simulink model "fs_driverless_top"  (R2026b)
settings: Solver=FixedStepDiscrete  StopTime=P.tEnd  FixedStep=P.dt
undefined symbols (not defined in the file): cones, lidarCfg, P, perception
libraries: sim3dlib x2, sim3dphyssensorlib x1, sim3dautolib x1
settings Model: Creator=User  LastModifiedBy=Jun Yee

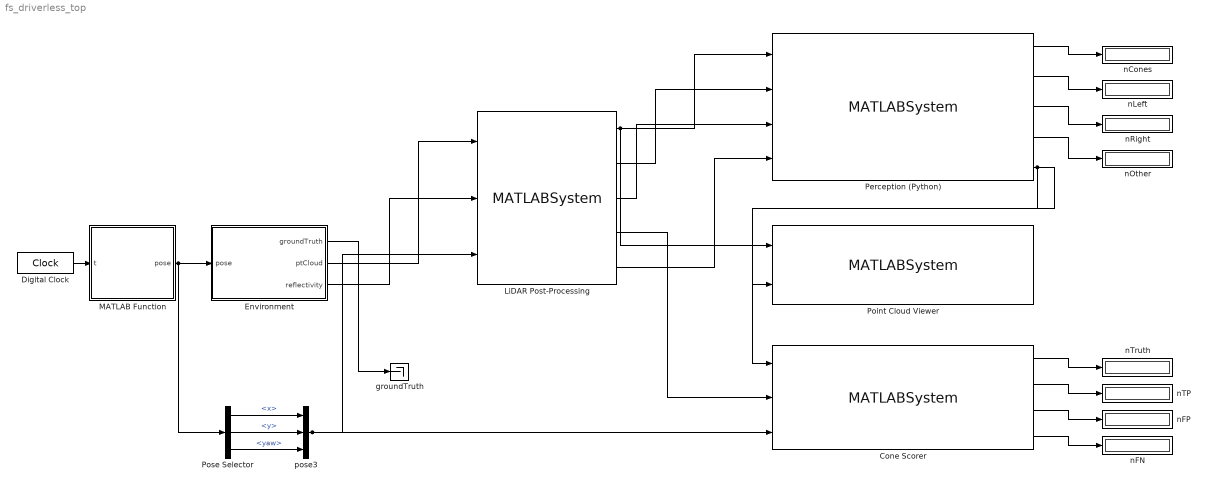
== system fs_driverless_top ==
  Cone Scorer : MATLABSystem  System=ConeScorer  MaxRange=P.score.maxRange  Gate=P.score.gate  MinHits=P.score.minHits  SensorOffset=lidarCfg.refToSensor  Ts=lidarCfg.Ts  PoseLag=lidarCfg.poseLagScans  SimulateUsing=Interpreted execution
      mask Type: ConeScorer
  Digital Clock : DigitalClock  SampleTime=P.dt
  Environment : Subsystem
  LiDAR Post-Processing : MATLABSystem  System=LidarPostProcess  MinRange=lidarCfg.minRange  MaxRange=lidarCfg.range  NoiseStd=lidarCfg.noiseStd  Ts=lidarCfg.Ts  Az=lidarCfg.az  ScanStartAz=lidarCfg.scanStartAz  SpinDir=lidarCfg.spinDir  SensorOffset=lidarCfg.refToSensor  Distortion=lidarCfg.motionDistortion  PoseLag=lidarCfg.poseLagScans  SimulateUsing=Interpreted execution
      mask Type: LidarPostProcess
  MATLAB Function : MATLAB Function  TreatAsAtomicUnit=on
  Perception (Python) : MATLABSystem  System=PerceptionPython  PythonFile=perception/perception.py  FunctionName=detect  MaxCones=150  Ts=lidarCfg.Ts  SimulateUsing=Interpreted execution
      mask Type: PerceptionPython
  Point Cloud Viewer : MATLABSystem  System=PointCloudViewer  XLim=[ -5, 40 ]  YLim=[ -20, 20 ]  ZLim=[ -1.5, 1.5 ]  GroundTol=0.04  ThinGround=4  SimulateUsing=Interpreted execution
      mask Type: PointCloudViewer
  Pose Selector : BusSelector  OutputSignals=x,y,yaw
  groundTruth : Terminator
  nCones : Display
  nFN : Display
  nFP : Display
  nLeft : Display
  nOther : Display
  nRight : Display
  nTP : Display
  nTruth : Display
  pose3 : Mux  Inputs=3
  wires:
  Digital Clock/1 -> MATLAB Function/1(t)
  MATLAB Function/1(pose) -> Environment/1(pose), Pose Selector/1
  Environment/1(groundTruth) -> groundTruth/1
  Environment/2(ptCloud) -> LiDAR Post-Processing/1
  Environment/3(reflectivity) -> LiDAR Post-Processing/2
  Pose Selector/1 -> pose3/1  "<x>"
  Pose Selector/2 -> pose3/2  "<y>"
  Pose Selector/3 -> pose3/3  "<yaw>"
  pose3/1 -> LiDAR Post-Processing/3, Cone Scorer/3
  LiDAR Post-Processing/1 -> Perception (Python)/1, Point Cloud Viewer/1
  LiDAR Post-Processing/2 -> Perception (Python)/2
  LiDAR Post-Processing/3 -> Perception (Python)/3
  LiDAR Post-Processing/5 -> Perception (Python)/4
  LiDAR Post-Processing/4 -> Cone Scorer/2
  Perception (Python)/5 -> Point Cloud Viewer/2, Cone Scorer/1
  Perception (Python)/1 -> nCones/1
  Perception (Python)/2 -> nLeft/1
  Perception (Python)/3 -> nRight/1
  Perception (Python)/4 -> nOther/1
  Cone Scorer/1 -> nTruth/1
  Cone Scorer/2 -> nTP/1
  Cone Scorer/3 -> nFP/1
  Cone Scorer/4 -> nFN/1

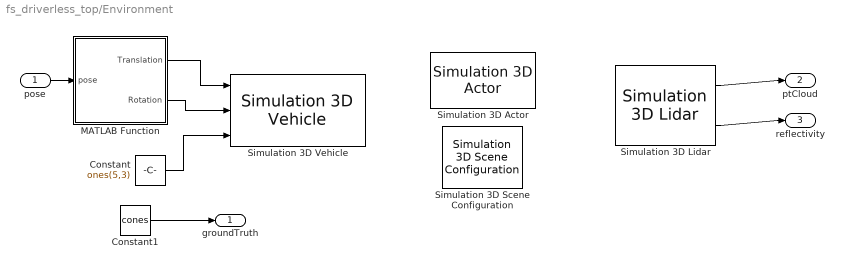
== system fs_driverless_top/Environment ==
  pose : Inport  OutDataTypeStr=Bus: VehiclePose
  Constant : Constant  Value=ones(5,3)
  Constant1 : Constant  Value=cones
  MATLAB Function : MATLAB Function  TreatAsAtomicUnit=on
  Simulation 3D Actor : sim3dlib/Simulation 3D Actor  Priority=1  ActorName=Cones  ParentName=Scene Origin  Operation=Create at setup  InitScriptText=|  SampleTime=-1  Translation=[0 0 0]  Rotation=[0 0 0]  Scale=[1 1 1]  aMode=aMode  ActorTag=Cones  ActorType=Sim3dActor  ID=C
      | % Flat ground plate the LiDAR can hit (the scene's own floor gives no LiDAR returns).
      | gnd = sim3d.Actor('ActorName', 'Ground');
      | createShape(gnd, 'box', [400 400 0.02]);
      | gnd.Translation = [0 0 -0.008];          % top face 2 mm above z = 0
      | gnd.Color = [0.3 0.3 0.3];
      | add(World, gnd, Actor);
      | 
      | try
      |     tn = evalin('base', 'P.trackName');
      | catch
      |     tn = 'autocross_01';
      | end
      | trackDir = fullfile(currentProject().RootFolder, 'tracks');
      | T = readtable(fullfile(trackDir, [tn '.csv']), 'TextType', 'string');
      | for k = 1:height(T)
      |     switch T.type(k)
      |         case "blue",         sz = [0.21 0.21 0.325]; col = [0 0.45 0.9];
      |         case "yellow",       sz = [0.21 0.21 0.325]; col = [1 0.8 0];
      |         case "orange_small", sz = [0.21 0.21 0.325]; col = [1 0.45 0];
      |         case "orange_big",   sz = [0.26 0.26 0.505]; col = [1 0.35 0];
      |         case "timekeeping",  sz = [0.30 0.30 1.20];  col = [0.8 0 0];
      |         otherwise,           sz = [0.21 0.21 0.60];  col = [0.5 0.5 0.5];
      |     end
      |     c = sim3d.Actor('ActorName', sprintf('Cone_%d', k));
      |     createShape(c, 'cone', sz);
      |     c.Translation = [T.x(k), -T.y(k), sz(3)/2];
      |     c.Color = col;
      |     add(World, c, Actor);
      | end
  Simulation 3D Lidar : sim3dphyssensorlib/Simulation 3D Lidar  Priority=1  sensorTag=Sim3dSensor  sensorId=1  sensorName=Pandar40P  vehTagList={'Custom ...';'Scene Origin';'SimulinkVehicle1'}  vehTag=SimulinkVehicle1  CoordinateSystem=ISO8855  mountLoc=Front bumper  offsetFlag=on  tmountOffset=lidarCfg.mountOffset  rmountOffset=[0 0 0]  DetectionRange=lidarCfg.range  RangeResolution=lidarCfg.rangeRes  FieldOfViewSpecification=Custom  VerticalFOV=40  VerticalFOVBounds=single([-55 15])  VerticalResolution=1.25  VerticalSampleAngles=lidarCfg.elev  HorizontalFOV=360  HorizontalFOVBounds=single([-180 180])  HorizontalResolution=0.16  HorizontalSampleAngles=lidarCfg.az  DistanceOutportEnabled=off  ReflectivityOutportEnabled=on  ReflectionModel=Phong  SemanticOutportEnabled=off  TransformOutportEnabled=off  SampleTime=lidarCfg.Ts  mountPoint=[0 0 0]  mountOrientation=[0 0 0]  aMode=3  ID=1
      settings: LibrarySourceBlock=drivingsim3d/Simulation 3D Lidar
  Simulation 3D Scene Configuration : sim3dlib/Simulation 3D Scene Configuration  Priority=0  ProjectFormat=Default Scenes  SceneDesc=Open surface  ProjectName=C:\Users\User\Documents\MATLAB\toolbox\shared\sim3d_projects\automotive_project_windows\UE\WindowsNoEditor\VehicleSimulation.exe  ScenePath=/Game/Maps/HwStrght  EnableOpenDRIVE=off  vehTagList={'Cones';'Custom';'Scene Origin';'SimulinkVehicle1'}  vehTag=SimulinkVehicle1  AttachedCameraRelativeTranslation=[0 0 0]  FreeCameraDefaultInitialTranslation=[-6, 0, 2]  AttachedCameraRelativeRotation=[0, -15, 0]  FreeCameraDefaultInitialRotation=[0, -15, 0]  ViewpointName=Custom  FreeCameraInitialTranslation=[0, 0, 0]  FreeCameraInitialRotation=[0, 0, 0]  OpVisEn=off  Ts=P.dt  EnableWindow=on  EnableRemoteAccess=off  SimulationMode=CoSimulation  SimulateUsing=Interpreted execution  EnableAnimationRecording=off  OverrideDefaultRecording=off  AnimationRecordingFileName=sim3dAnimation.mat  AnimationRecordingInterval=[0 inf]  EnableWeather=off  SunAzimuth=90  SunAltitude=40.0  EnableGeospatialSun=off  Latitude=0  Longitude=0  Date=2023-01-01  Time=10:30:00  GeoTimeZone=-5.0  SunDaylightSaving=off  wind=1  clouds=10  EnableVolumetricClouds=off  CloudCoverage=0  CloudAltitude=6  fog=0  rain=0  RaindropsEffect=off  SnowDensity=0  EnableGeospatial=off  TilesetSource=Earth terrain  UseTrueOrigin=off  OriginHeight=200  OriginLatitude=40.744652  OriginLongitude=-73.988864  MapStyle=Aerial  AdditionalAssetIDs=[]  UseAdvancedSunSky=off  SolarTime=11  TimeZone=-5  Day=21  Month=9  Year=2022  UseDaylightSavingTime=on  DSTStartDay=10  DSTStartMonth=3  DSTEndDay=3  DSTEndMonth=11  DSTSwitchHour=2  sensorTag=MainCamera1  sensorId=1  sensorName=MainCamera1  mountLoc=Origin  offsetFlag=off  tmountOffset=[0, 0, 0]  rmountOffset=[0, 0, 0]  HorizontalResolution=1280  VerticalResolution=720  HorizontalFOV=60  mountPoint=[0 0 0]  mountOrientation=[0 0 0]  aMode=3  ID=1  GeoTrigger=Inactive  ViewNameList={'Custom'}  ViewTranslationList={'[0 0 0]'}  ViewRotationList={'[0 0 0]'}
      settings: LibrarySourceBlock=drivingsim3d/Simulation 3D Scene Configuration
  Simulation 3D Vehicle : sim3dautolib/Simulation 3D Vehicle  Priority=-1  PassVehMesh=Formula student vehicle  MeshPath=/MathWorksAutomotiveContent/Vehicles/Muscle/Meshes/SK_MuscleCar.SK_MuscleCar  VehColor=Blue  ActorName=SimulinkVehicle1  VehLightsControl=off  HeadlightColor=[ 1, 1, 1 ]  HighBeamIntensity=100000  LowBeamIntensity=60000  HighBeamConeAngle=1.22  LowBeamConeAngle=1.22  LeftHeadlightOrientation=[ 0, 0 ]  RightHeadlightOrientation=[ 0, 0 ]  BrakelightIntensity=500  ReverselightIntensity=500  SignallightIntensity=500  SignallightPeriod=1  SignalPulseWidth=50  Translation=zeros( 5, 3 )  Rotation=zeros( 5, 3 )  Scale=ones( 5, 3 )  SampleTime=-1  ActorType=SimulinkVehicle  ID=1  aMode=2  ActorTag=SimulinkVehicle1
      settings: LibrarySourceBlock=vehdynlibsim3d/Simulation 3D Vehicle
  groundTruth : Outport
  ptCloud : Outport  Port=2
  reflectivity : Outport  Port=3
  wires:
  Constant1/1 -> groundTruth/1
  pose/1 -> MATLAB Function/1(pose)
  MATLAB Function/1(Translation) -> Simulation 3D Vehicle/1
  MATLAB Function/2(Rotation) -> Simulation 3D Vehicle/2
  Constant/1 -> Simulation 3D Vehicle/3
  Simulation 3D Lidar/1 -> ptCloud/1
  Simulation 3D Lidar/2 -> reflectivity/1

== matlab function fs_driverless_top/Environment/MATLAB Function ==
  data: pose input Bus: VehiclePose; Translation output; Rotation output
function [Translation, Rotation] = PoseToSim3D(pose)
% Convert our pose (y left, yaw anticlockwise, rad) to the SAE
% convention used by the Vehicle Dynamics Blockset 3D vehicle
% (y right, z down, yaw clockwise). Row 1 = car body, rows 2-5 = wheels.
Translation = zeros(5, 3);
Rotation    = zeros(5, 3);
Translation(1, :) = [pose.x, -pose.y, 0];
Rotation(1, 3)    = -pose.yaw;

== matlab function fs_driverless_top/MATLAB Function ==
  data: t input; testDrive parameter; pose output Bus: VehiclePose
   function pose  = TestDriver(t, testDrive)
   % TEMPORARY: moves the car along the true centreline at constant speed.
   % Stand-in for Vehicle dynamics, for testing the Environment only.
   N = size(testDrive.centre, 1);
   i = floor(testDrive.speed * t / testDrive.ds) + 1;
   if testDrive.closed > 0
       i  = mod(i - 1, N) + 1;
       i2 = mod(i + 3, N) + 1;
   else
       i  = min(i, N - 4);
       i2 = i + 4;
   end
   p = testDrive.centre(i, :);
   d = testDrive.centre(i2, :) - p;
   pose.x = p(1);  pose.y = p(2);  pose.z = 0;
   pose.roll = 0;  pose.pitch = 0;
   pose.yaw = atan2(d(2), d(1));
